simulink model "INDI_Rate_Controller_Example"  (R2018b)
settings: Solver=ode4  StartTime=0.0  StopTime=5  FixedStep=0.001  RelTol=1e-3
values from neighbouring files (symbols this model uses):
  omega_actuator = 80    [INDI_Rate_Controller_Example_init.m]
  omega_filter = 100    [INDI_Rate_Controller_Example_init.m]
  omega_reference = 10    [INDI_Rate_Controller_Example_init.m]
undefined symbols (not defined in the file or in its folder): INDI_cntrl, K_p, ss_model
settings Model: Creator=Fgücker  LastModifiedBy=yannic

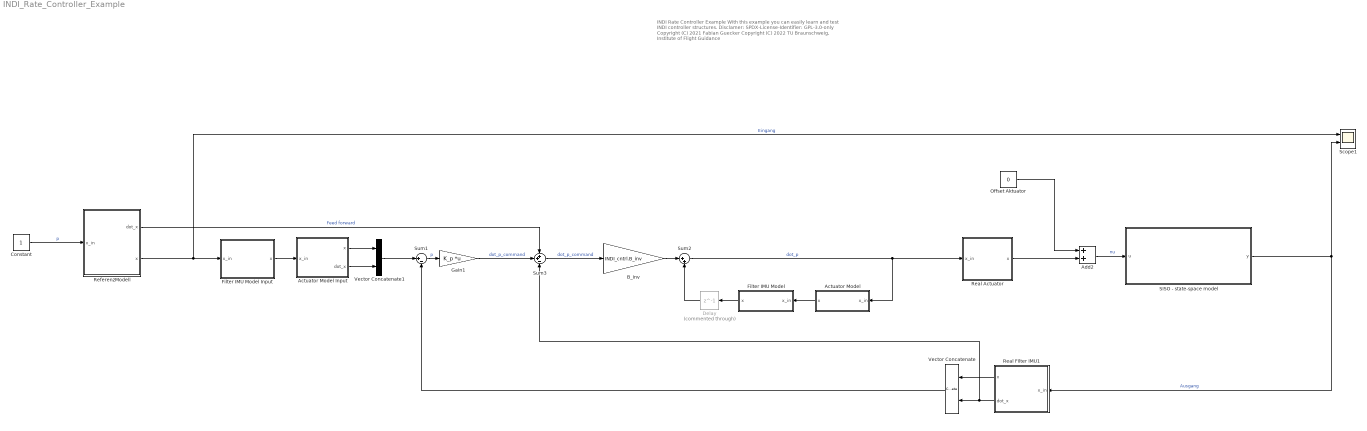
== system INDI_Rate_Controller_Example ==
  note: INDI Rate Controller Example
      |
      | With this example you can easily learn and test INDI controller structures.
      |
      | Disclamer:
      | SPDX-License-Identifier: GPL-3.0-only
      |
      | Copyright (C) 2021 Fabian Guecker
      | Copyright (C) 2022 TU Braunschweig, Institute of Flight Guidance
  Actuator Model : Subsystem  mask{omega=omega_actuator, D=1, ref_pos=0}
      mask prompts: ref_pos "Inital Position"
  Actuator Model Input : Subsystem  mask{omega=omega_actuator, D=1, ref_pos=0}
      mask prompts: ref_pos "Inital Position"
  Add2 : Sum
  B_inv : Gain  Gain=INDI_cntrl.B_inv
  Constant : Constant
  Delay : Delay  Commented=through  DelayLength=1
  Filter IMU Model : Subsystem  mask{omega=omega_filter, D=1, ref_pos=0}
      mask prompts: ref_pos "Inital Position"
  Filter IMU Model Input : Subsystem  mask{omega=omega_filter, D=1, ref_pos=0}
      mask prompts: ref_pos "Inital Position"
  Gain1 : Gain  Gain=K_p  Multiplication=Matrix(K*u)
  Offset Aktuator : Constant  Value=0
  Real Actuator : Subsystem  mask{omega=omega_actuator, D=1, ref_pos=0}
      mask prompts: ref_pos "Inital Position"
  Real Filter IMU1 : Subsystem  mask{omega=omega_filter, D=1, ref_pos=0}
      mask prompts: ref_pos "Inital Position"
  ReferenzModell : Subsystem  mask{omega=omega_reference, D=1, ref_pos=0}
      mask prompts: ref_pos "Inital Position"
  SISO - state-space model : Subsystem
  Scope1 : Scope  NumInputPorts=2
  Sum1 : Sum  Inputs=|+-
  Sum2 : Sum  Inputs=|++
  Sum3 : Sum  Inputs=++-
  Vector Concatenate : Concatenate
  Vector Concatenate1 : Concatenate
  wires:
  Sum1/1 -> Gain1/1  "p"
  Sum3/1 -> B_inv/1  "dot_p_command"
  B_inv/1 -> Sum2/1
  Sum2/1 -> Actuator Model/1(x_in), Real Actuator/1(x_in)  "dot_p"
  Delay/1 -> Sum2/2
  SISO - state-space model/1(y) -> Real Filter IMU1/1(x_in), Scope1/2  "Ausgang"
  Constant/1 -> ReferenzModell/1(x_in)  "p"
  Filter IMU Model/1(x) -> Delay/1
  ReferenzModell/2(x) -> Scope1/1, Filter IMU Model Input/1(x_in)  "Eingang"
  Gain1/1 -> Sum3/2  "dot_p_command"
  Real Filter IMU1/2(dot_x) -> Sum3/3, Vector Concatenate/2
  Add2/1 -> SISO - state-space model/1(u)  "nu"
  Real Actuator/1(x) -> Add2/2
  Offset Aktuator/1 -> Add2/1
  Filter IMU Model Input/1(x) -> Actuator Model Input/1(x_in)
  Real Filter IMU1/1(x) -> Vector Concatenate/1
  Actuator Model/1(x) -> Filter IMU Model/1(x_in)
  Actuator Model Input/1(x) -> Vector Concatenate1/1
  Vector Concatenate1/1 -> Sum1/1
  Vector Concatenate/1 -> Sum1/2
  Actuator Model Input/2(dot_x) -> Vector Concatenate1/2
  ReferenzModell/1(dot_x) -> Sum3/1  "Feed forward"

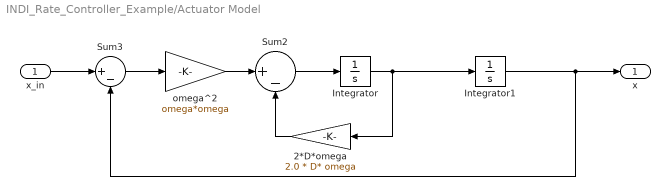
== system INDI_Rate_Controller_Example/Actuator Model ==
  x_in : Inport
  2*D*omega : Gain  Gain=2.0 * D* omega  SaturateOnIntegerOverflow=on  OutDataTypeStr=Inherit: Same as input  ParamDataTypeStr=Inherit: Same as input
  Integrator : Integrator
  Integrator1 : Integrator
  Sum2 : Sum  Inputs=|+-  SaturateOnIntegerOverflow=on  InputSameDT=on  OutDataTypeStr=Inherit: Same as first input
  Sum3 : Sum  Inputs=|+-  SaturateOnIntegerOverflow=on  InputSameDT=on  OutDataTypeStr=Inherit: Same as first input
  omega^2 : Gain  Gain=omega*omega  SaturateOnIntegerOverflow=on  OutDataTypeStr=Inherit: Same as input  ParamDataTypeStr=Inherit: Same as input
  x : Outport  InitialOutput=0
  wires:
  Integrator/1 -> Integrator1/1, 2*D*omega/1
  Sum2/1 -> Integrator/1
  x_in/1 -> Sum3/1
  Sum3/1 -> omega^2/1
  Integrator1/1 -> x/1, Sum3/2
  omega^2/1 -> Sum2/1
  2*D*omega/1 -> Sum2/2

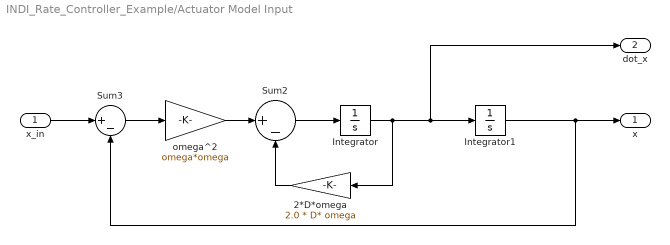
== system INDI_Rate_Controller_Example/Actuator Model Input ==
  x_in : Inport
  2*D*omega : Gain  Gain=2.0 * D* omega  SaturateOnIntegerOverflow=on  OutDataTypeStr=Inherit: Same as input  ParamDataTypeStr=Inherit: Same as input
  Integrator : Integrator
  Integrator1 : Integrator
  Sum2 : Sum  Inputs=|+-  SaturateOnIntegerOverflow=on  InputSameDT=on  OutDataTypeStr=Inherit: Same as first input
  Sum3 : Sum  Inputs=|+-  SaturateOnIntegerOverflow=on  InputSameDT=on  OutDataTypeStr=Inherit: Same as first input
  omega^2 : Gain  Gain=omega*omega  SaturateOnIntegerOverflow=on  OutDataTypeStr=Inherit: Same as input  ParamDataTypeStr=Inherit: Same as input
  x : Outport  InitialOutput=0
  dot_x : Outport  Port=2  InitialOutput=0
  wires:
  Integrator/1 -> dot_x/1, Integrator1/1, 2*D*omega/1
  Sum2/1 -> Integrator/1
  x_in/1 -> Sum3/1
  Sum3/1 -> omega^2/1
  Integrator1/1 -> x/1, Sum3/2
  omega^2/1 -> Sum2/1
  2*D*omega/1 -> Sum2/2

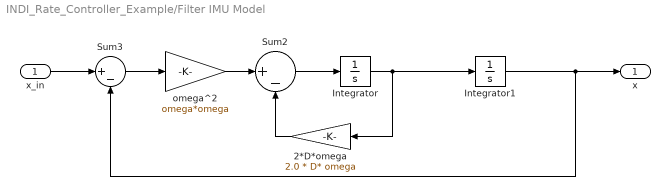
== system INDI_Rate_Controller_Example/Filter IMU Model ==
  x_in : Inport
  2*D*omega : Gain  Gain=2.0 * D* omega  SaturateOnIntegerOverflow=on  OutDataTypeStr=Inherit: Same as input  ParamDataTypeStr=Inherit: Same as input
  Integrator : Integrator
  Integrator1 : Integrator
  Sum2 : Sum  Inputs=|+-  SaturateOnIntegerOverflow=on  InputSameDT=on  OutDataTypeStr=Inherit: Same as first input
  Sum3 : Sum  Inputs=|+-  SaturateOnIntegerOverflow=on  InputSameDT=on  OutDataTypeStr=Inherit: Same as first input
  omega^2 : Gain  Gain=omega*omega  SaturateOnIntegerOverflow=on  OutDataTypeStr=Inherit: Same as input  ParamDataTypeStr=Inherit: Same as input
  x : Outport  InitialOutput=0
  wires:
  Integrator/1 -> Integrator1/1, 2*D*omega/1
  Sum2/1 -> Integrator/1
  x_in/1 -> Sum3/1
  Sum3/1 -> omega^2/1
  Integrator1/1 -> x/1, Sum3/2
  omega^2/1 -> Sum2/1
  2*D*omega/1 -> Sum2/2

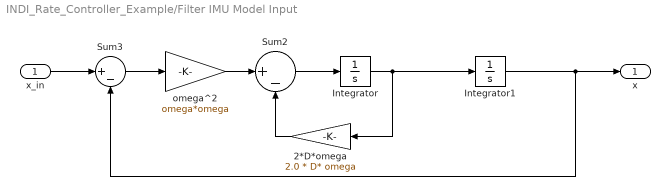
== system INDI_Rate_Controller_Example/Filter IMU Model Input ==
  x_in : Inport
  2*D*omega : Gain  Gain=2.0 * D* omega  SaturateOnIntegerOverflow=on  OutDataTypeStr=Inherit: Same as input  ParamDataTypeStr=Inherit: Same as input
  Integrator : Integrator
  Integrator1 : Integrator  InitialCondition=ref_pos
  Sum2 : Sum  Inputs=|+-  SaturateOnIntegerOverflow=on  InputSameDT=on  OutDataTypeStr=Inherit: Same as first input
  Sum3 : Sum  Inputs=|+-  SaturateOnIntegerOverflow=on  InputSameDT=on  OutDataTypeStr=Inherit: Same as first input
  omega^2 : Gain  Gain=omega*omega  SaturateOnIntegerOverflow=on  OutDataTypeStr=Inherit: Same as input  ParamDataTypeStr=Inherit: Same as input
  x : Outport  InitialOutput=0
  wires:
  Integrator/1 -> Integrator1/1, 2*D*omega/1
  Sum2/1 -> Integrator/1
  x_in/1 -> Sum3/1
  Sum3/1 -> omega^2/1
  Integrator1/1 -> x/1, Sum3/2
  omega^2/1 -> Sum2/1
  2*D*omega/1 -> Sum2/2

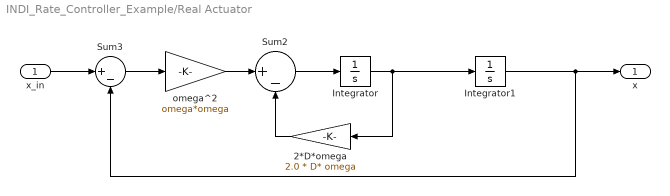
== system INDI_Rate_Controller_Example/Real Actuator ==
  x_in : Inport
  2*D*omega : Gain  Gain=2.0 * D* omega  SaturateOnIntegerOverflow=on  OutDataTypeStr=Inherit: Same as input  ParamDataTypeStr=Inherit: Same as input
  Integrator : Integrator
  Integrator1 : Integrator
  Sum2 : Sum  Inputs=|+-  SaturateOnIntegerOverflow=on  InputSameDT=on  OutDataTypeStr=Inherit: Same as first input
  Sum3 : Sum  Inputs=|+-  SaturateOnIntegerOverflow=on  InputSameDT=on  OutDataTypeStr=Inherit: Same as first input
  omega^2 : Gain  Gain=omega*omega  SaturateOnIntegerOverflow=on  OutDataTypeStr=Inherit: Same as input  ParamDataTypeStr=Inherit: Same as input
  x : Outport  InitialOutput=0
  wires:
  Integrator/1 -> Integrator1/1, 2*D*omega/1
  Sum2/1 -> Integrator/1
  x_in/1 -> Sum3/1
  Sum3/1 -> omega^2/1
  Integrator1/1 -> x/1, Sum3/2
  omega^2/1 -> Sum2/1
  2*D*omega/1 -> Sum2/2

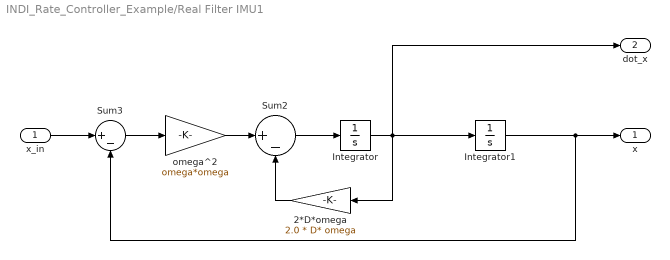
== system INDI_Rate_Controller_Example/Real Filter IMU1 ==
  x_in : Inport
  2*D*omega : Gain  Gain=2.0 * D* omega  SaturateOnIntegerOverflow=on  OutDataTypeStr=Inherit: Same as input  ParamDataTypeStr=Inherit: Same as input
  Integrator : Integrator
  Integrator1 : Integrator
  Sum2 : Sum  Inputs=|+-  SaturateOnIntegerOverflow=on  InputSameDT=on  OutDataTypeStr=Inherit: Same as first input
  Sum3 : Sum  Inputs=|+-  SaturateOnIntegerOverflow=on  InputSameDT=on  OutDataTypeStr=Inherit: Same as first input
  omega^2 : Gain  Gain=omega*omega  SaturateOnIntegerOverflow=on  OutDataTypeStr=Inherit: Same as input  ParamDataTypeStr=Inherit: Same as input
  x : Outport  InitialOutput=0
  dot_x : Outport  Port=2  InitialOutput=0
  wires:
  Integrator/1 -> dot_x/1, Integrator1/1, 2*D*omega/1
  Sum2/1 -> Integrator/1
  x_in/1 -> Sum3/1
  Sum3/1 -> omega^2/1
  Integrator1/1 -> x/1, Sum3/2
  omega^2/1 -> Sum2/1
  2*D*omega/1 -> Sum2/2

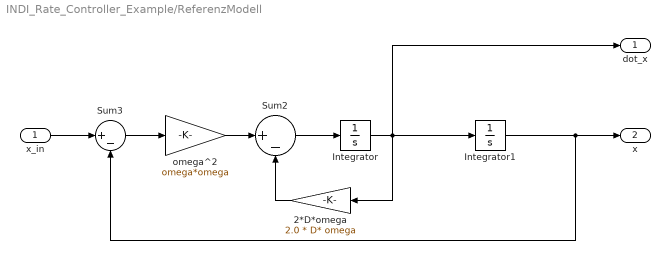
== system INDI_Rate_Controller_Example/ReferenzModell ==
  x_in : Inport
  2*D*omega : Gain  Gain=2.0 * D* omega  SaturateOnIntegerOverflow=on  OutDataTypeStr=Inherit: Same as input  ParamDataTypeStr=Inherit: Same as input
  Integrator : Integrator
  Integrator1 : Integrator  InitialCondition=ref_pos
  Sum2 : Sum  Inputs=|+-  SaturateOnIntegerOverflow=on  InputSameDT=on  OutDataTypeStr=Inherit: Same as first input
  Sum3 : Sum  Inputs=|+-  SaturateOnIntegerOverflow=on  InputSameDT=on  OutDataTypeStr=Inherit: Same as first input
  omega^2 : Gain  Gain=omega*omega  SaturateOnIntegerOverflow=on  OutDataTypeStr=Inherit: Same as input  ParamDataTypeStr=Inherit: Same as input
  dot_x : Outport  InitialOutput=0
  x : Outport  Port=2  InitialOutput=0
  wires:
  Integrator/1 -> dot_x/1, Integrator1/1, 2*D*omega/1
  Sum2/1 -> Integrator/1
  x_in/1 -> Sum3/1
  Sum3/1 -> omega^2/1
  Integrator1/1 -> x/1, Sum3/2
  omega^2/1 -> Sum2/1
  2*D*omega/1 -> Sum2/2

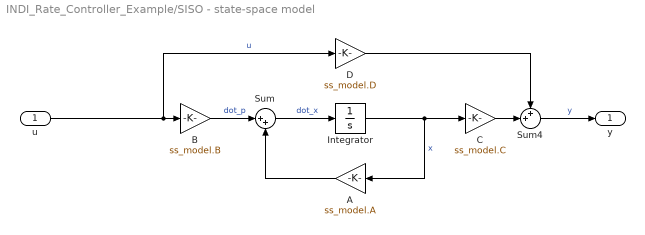
== system INDI_Rate_Controller_Example/SISO - state-space model ==
  u : Inport
  A : Gain  Gain=ss_model.A
  B : Gain  Gain=ss_model.B
  C : Gain  Gain=ss_model.C
  D : Gain  Gain=ss_model.D
  Integrator : Integrator
  Sum : Sum  Inputs=|++
  Sum4 : Sum  Inputs=++|
  y : Outport
  wires:
  Sum4/1 -> y/1  "y"
  B/1 -> Sum/1  "dot_p"
  u/1 -> D/1, B/1  "u"
  D/1 -> Sum4/1
  C/1 -> Sum4/2
  Sum/1 -> Integrator/1  "dot_x"
  Integrator/1 -> C/1, A/1  "x"
  A/1 -> Sum/2
